simulink model "kol_model"  (R2026b)
settings: Solver=ode4  StopTime=T  FixedStep=dt
values from neighbouring files (symbols this model uses):
  S = sim_param(q, D(k).ac, kp)    [deney_4a.m]    (also in dogrula_2.m = sim_param(q, h.ac, ref.kp); dogrula_3.m = sim_param(q, h.ac, kp); dogrula_b2.m = sim_param(q, ac, kp); dogrula_b2_dt.m = sim_param(q, ac, kp))
settings Model: Creator=safak  LastModifiedBy=safak
settings DataIOCC: Decimation=dec  SaveTime=off  SignalLogging=off

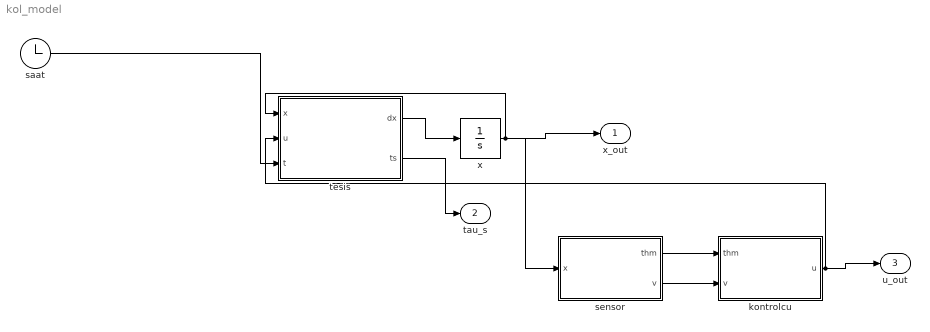
== system kol_model ==
  kontrolcu : MATLAB Function  TreatAsAtomicUnit=on
  saat : Clock
  sensor : MATLAB Function  TreatAsAtomicUnit=on
  tesis : MATLAB Function  TreatAsAtomicUnit=on
  x : Integrator  InitialCondition=S.x0
  x_out : Outport
  tau_s : Outport  Port=2
  u_out : Outport  Port=3
  wires:
  x/1 -> tesis/1(x), x_out/1, sensor/1(x)
  kontrolcu/1(u) -> tesis/2(u), u_out/1
  saat/1 -> tesis/3(t)
  tesis/1(dx) -> x/1
  tesis/2(ts) -> tau_s/1
  sensor/1(thm) -> kontrolcu/1(thm)
  sensor/2(v) -> kontrolcu/2(v)

== matlab function kol_model/sensor ==
  settings: updateMethod=DISCRETE  sampleTime=Ts
  data: x input; thm output; v output; S parameter
function [thm, v] = sensor(x, S)
% Kol açısı ölçümü (nicemleme + gL örnek gecikme) ve hız (gerçek ya da kestirilmiş).
% kol_benzetim.m'deki kontrolcü örneğinin ölçüm kısmı ile aynı sıra.
persistent buf vhat yprev
vi = 3;  qv = S.qL;
if S.motorD > 0, vi = 1;  qv = S.qM; end
if isempty(buf)
    buf = olc(x(3), S.qL)*ones(21,1);
    yprev = olc(x(vi), qv);
    vhat = 0;
end
thm = olc(x(3), S.qL);
if S.gL > 0
    buf = [buf(2:end); thm];
    thm = buf(21 - S.gL);
end
if S.fv_inf > 0
    v = x(vi + 1);
else
    yv = olc(x(vi), qv);
    vhat = vhat + S.aV*((yv - yprev)/S.Ts - vhat);
    yprev = yv;
    v = vhat;
end
end

function y = olc(x, q)
y = x;
if q > 0, y = q*floor(x/q); end
end

== matlab function kol_model/tesis ==
  data: x input; u input; dx output; t input; ts output; S parameter
function [dx, ts] = tesis(x, u, t, S)
% İki kütle + dişli teması (kol tarafına indirgenmiş). kol_benzetim.m / f(x) ile aynı.
phi = x(1);  dphi = x(2);  th = x(3);  dth = x(4);
d = phi - th;  dd = dphi - dth;
ts = 0;
if d > S.r
    ts = max(S.Ks*(d - S.r) + S.cs*dd, 0);     % temas yalnız iter, çekmez
elseif d < -S.r
    ts = min(S.Ks*(d + S.r) + S.cs*dd, 0);
end
tf = 0;
if S.Fc > 0                                    % yumuşatılmış Stribeck sürtünmesi
    tf = (S.Fc + (S.Fs - S.Fc)*exp(-(dphi/S.vs)^2)) * tanh(dphi/S.veps);
end
bz = 0;
if t < S.dT
    bz = S.dA*sin(2*pi*S.df*t);                % yük bozucusu
end
dx = [dphi;
      (u - S.bM*dphi - tf - ts)/S.JM;
      dth;
      (ts - S.bL*dth - S.mgl*sin(th) + bz)/S.JL];
end

== matlab function kol_model/kontrolcu ==
  settings: updateMethod=DISCRETE  sampleTime=Ts
  data: thm input; u output; v input; S parameter
function u = kontrolcu(thm, v, S)
% PID ya da P-PI kaskat + tork sınırı + basit anti-windup + sürücü ölü bandı.
persistent z
if isempty(z), z = S.z0; end
e = S.ref - thm;
if S.ppi > 0
    ev = S.kp*e - v;                 % hız hatası (kol tarafı)
    u0 = S.KV*ev + S.KI*z;
    iz = ev;
else
    u0 = S.Kp*e + S.Ki*z - S.Kd*v;
    iz = e;
end
u = min(max(u0, -S.Tmax), S.Tmax);
doy = (u0 > S.Tmax && iz > 0) || (u0 < -S.Tmax && iz < 0);
if ~doy, z = z + iz*S.Ts; end
if abs(u) < S.olu, u = 0; end
end
